simulink model "sensor_real_corriente_LU"  (R2026b)
settings: Solver=VariableStepAuto
values from neighbouring files (symbols this model uses):
  wn_I = 6000    [coeficientes.m]
  zeta_I = 1    [coeficientes.m]
settings Model: Creator=lamun  LastModifiedBy=lamun

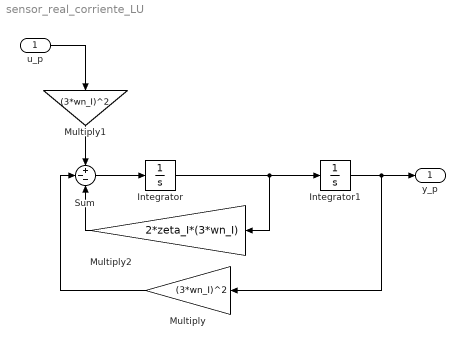
== system sensor_real_corriente_LU ==
  u_p : Inport
  Integrator : Integrator
  Integrator1 : Integrator
  Multiply : Gain  Gain=(3*wn_I)^2
  Multiply1 : Gain  Gain=(3*wn_I)^2
  Multiply2 : Gain  Gain=2*zeta_I*(3*wn_I)
  Sum : Sum  Inputs=+--
  y_p : Outport
  wires:
  Integrator/1 -> Multiply2/1, Integrator1/1
  Multiply1/1 -> Sum/1
  u_p/1 -> Multiply1/1
  Multiply2/1 -> Sum/3
  Sum/1 -> Integrator/1
  Multiply/1 -> Sum/2
  Integrator1/1 -> Multiply/1, y_p/1
